simulink model "Cable_Wo_M_Inductance_Modelling_Study"  (R2024b)
settings: Solver=FixedStepDiscrete  StartTime=0.0  StopTime=5  FixedStep=1e-6  RelTol=1e-3  AbsTol=1
values from neighbouring files (symbols this model uses):
  Ccs1 = 733.62e-12    (= 7.3362e-10)    [Cable_Data_Inductance_Study.m]
  Ccs2 = 733.62e-12    (= 7.3362e-10)    [Cable_Data_Inductance_Study.m]
  Lc1 = 0.092e-6    (= 9.2e-08)    [Cable_Data_Inductance_Study.m]
  Lc1_total = Lc1 + Mcs1    (= 2.72e-07)    [Cable_Data_Inductance_Study.m]
  Lc2 = 0.092e-6    (= 9.2e-08)    [Cable_Data_Inductance_Study.m]
  Lc2_total = Lc2 + Mcs2    (= 2.72e-07)    [Cable_Data_Inductance_Study.m]
  Len35_batt1_HVJB1_neg = 0.600    (= 0.6)    [Cable_Data_Inductance_Study.m]
  Len35_batt1_HVJB1_pos = 0.750    (= 0.75)    [Cable_Data_Inductance_Study.m]
  Ls1_eff = Ls1 + Mss_cal    [Cable_Data_Inductance_Study.m]
  Ls2_eff = Ls2 + Mss_cal    [Cable_Data_Inductance_Study.m]
  Rc1 = 0.38e-3    (= 0.00038)    [Cable_Data_Inductance_Study.m]
  Rc2 = 0.38e-3    (= 0.00038)    [Cable_Data_Inductance_Study.m]
  Rs1 = 2.55e-3    (= 0.00255)    [Cable_Data_Inductance_Study.m]
  Rs2 = 2.55e-3    (= 0.00255)    [Cable_Data_Inductance_Study.m]
undefined symbols (not defined in the file or in its folder): DiscIntNeverNeededParam, Lns95, Lps95
libraries: spsSeriesRLCBranchLib x59, spsCurrentMeasurementLib x12, spsVoltageMeasurementLib x9, spsGroundLib x6, spsMultimeterLib x6, eeGeneralControl x2, spsVariableResistorLib x2, spsDCVoltageSourceLib x2, spspowerguiLib x1, sps_lib x1
(part 2 of 2)

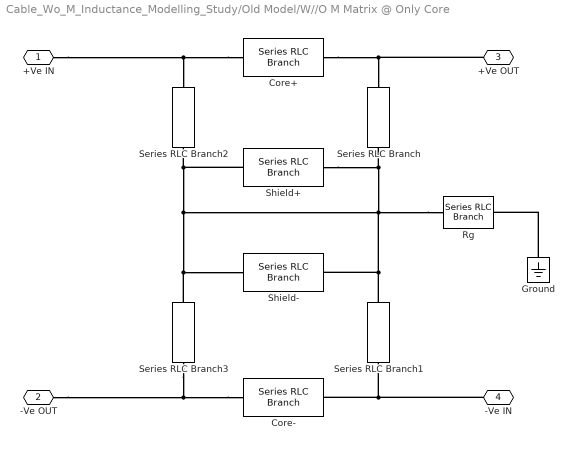
== system Cable_Wo_M_Inductance_Modelling_Study/Old Model/W//O M Matrix @ Only Core ==
  Core+ : spsSeriesRLCBranchLib/Series RLC Branch  LConnTagsString=__new0  RConnTagsString=__new0  BranchType=RL  Resistance=Rc1*Len35_batt1_HVJB1_pos  Inductance=Lc1_total*Len35_batt1_HVJB1_pos  SetiL0=off  InitialCurrent=0  Capacitance=1e-6  Setx0=off  InitialVoltage=0  Measurements=Branch voltage and current
  Core- : spsSeriesRLCBranchLib/Series RLC Branch  LConnTagsString=__new0  RConnTagsString=__new0  BranchType=RL  Resistance=Rc2*Len35_batt1_HVJB1_neg  Inductance=Lc2_total*Len35_batt1_HVJB1_neg  SetiL0=off  InitialCurrent=0  Capacitance=1e-6  Setx0=off  InitialVoltage=0  Measurements=Branch voltage and current
  Ground : spsGroundLib/Ground  LConnTagsString=a
  Rg : spsSeriesRLCBranchLib/Series RLC Branch  LConnTagsString=__new0  RConnTagsString=__new0  BranchType=R  Resistance=10e-03  Inductance=1e-3  SetiL0=off  InitialCurrent=0  Capacitance=1e-6  Setx0=off  InitialVoltage=0  Measurements=Branch voltage and current
  Series RLC Branch : spsSeriesRLCBranchLib/Series RLC Branch  LConnTagsString=__new0  RConnTagsString=__new0  BranchType=C  Resistance=1  Inductance=1e-3  SetiL0=off  InitialCurrent=0  Capacitance=(Ccs1/2)*Len35_batt1_HVJB1_pos  Setx0=off  InitialVoltage=0  Measurements=None
  Series RLC Branch1 : spsSeriesRLCBranchLib/Series RLC Branch  LConnTagsString=__new0  RConnTagsString=__new0  BranchType=C  Resistance=1  Inductance=1e-3  SetiL0=off  InitialCurrent=0  Capacitance=(Ccs2/2)*Len35_batt1_HVJB1_neg  Setx0=off  InitialVoltage=0  Measurements=None
  Series RLC Branch2 : spsSeriesRLCBranchLib/Series RLC Branch  LConnTagsString=__new0  RConnTagsString=__new0  BranchType=C  Resistance=1  Inductance=1e-3  SetiL0=off  InitialCurrent=0  Capacitance=(Ccs1/2)*Len35_batt1_HVJB1_pos  Setx0=off  InitialVoltage=0  Measurements=None
  Series RLC Branch3 : spsSeriesRLCBranchLib/Series RLC Branch  LConnTagsString=__new0  RConnTagsString=__new0  BranchType=C  Resistance=1  Inductance=1e-3  SetiL0=off  InitialCurrent=0  Capacitance=(Ccs2/2)*Len35_batt1_HVJB1_neg  Setx0=off  InitialVoltage=0  Measurements=None
  Shield+ : spsSeriesRLCBranchLib/Series RLC Branch  LConnTagsString=__new0  RConnTagsString=__new0  BranchType=R  Resistance=Rs1*Len35_batt1_HVJB1_pos  Inductance=Lps95*3.270  SetiL0=off  InitialCurrent=0  Capacitance=1e-6  Setx0=off  InitialVoltage=0  Measurements=Branch voltage and current
  Shield- : spsSeriesRLCBranchLib/Series RLC Branch  LConnTagsString=__new0  RConnTagsString=__new0  BranchType=R  Resistance=Rs2*Len35_batt1_HVJB1_neg  Inductance=Lns95*3.305  SetiL0=off  InitialCurrent=0  Capacitance=1e-6  Setx0=off  InitialVoltage=0  Measurements=Branch voltage and current
  +Ve IN : PMIOPort  Side=Left
  -Ve OUT : PMIOPort  Port=2  Side=Left
  +Ve OUT : PMIOPort  Port=3  Side=Right
  -Ve IN : PMIOPort  Port=4  Side=Right
  connections:
  Core-/RConn1 -- Series RLC Branch1/LConn1 -- -Ve IN/RConn1
  Rg/LConn1 -- Series RLC Branch2/RConn1 -- Shield+/LConn1 -- Shield-/LConn1 -- Series RLC Branch3/RConn1 -- Shield-/RConn1 -- Series RLC Branch1/RConn1 -- Shield+/RConn1 -- Series RLC Branch/RConn1
  Core+/RConn1 -- +Ve OUT/RConn1 -- Series RLC Branch/LConn1
  Core+/LConn1 -- +Ve IN/RConn1 -- Series RLC Branch2/LConn1
  Ground/LConn1 -- Rg/RConn1
  Core-/LConn1 -- -Ve OUT/RConn1 -- Series RLC Branch3/LConn1

== system Cable_Wo_M_Inductance_Modelling_Study/Old Model/Constant Aux Load 100A/DC Link Capacitor ==
  Current Measurement1 : spsCurrentMeasurementLib/Current Measurement  PhasorSimulation=off  OutputType=Complex  PSBequivalent=0
  Cx : spsSeriesRLCBranchLib/Series RLC Branch  LConnTagsString=__new0  RConnTagsString=__new0  BranchType=C  Resistance=0.5  Inductance=1e-3  SetiL0=off  InitialCurrent=0  Capacitance=2e-3  Setx0=on  InitialVoltage=Cx_Vs  Measurements=Branch voltage and current
  To Workspace1 : ToWorkspace  VariableName=DCLinkCapVoltage  SaveFormat=Timeseries  SampleTime=-1
  To Workspace2 : ToWorkspace  VariableName=DCLinkCapCurrent  SaveFormat=Timeseries  SampleTime=-1
  Voltage Measurement : spsVoltageMeasurementLib/Voltage Measurement  PhasorSimulation=off  OutputType=Complex  PSBequivalent=0
  + : PMIOPort  Side=Left
  - : PMIOPort  Port=2  Side=Right
  wires:
  Voltage Measurement/1 -> To Workspace1/1
  Current Measurement1/1 -> To Workspace2/1
  connections:
  Current Measurement1/RConn1 -- -/RConn1 -- Voltage Measurement/LConn2
  Cx/RConn1 -- Current Measurement1/LConn1
  Voltage Measurement/LConn1 -- +/RConn1 -- Cx/LConn1
